simulink model "trajgen"  (Simulink 4.00)
settings: Solver=ode45  StartTime=0.0  StopTime=10.0  RelTol=1e-3
undefined symbols (not defined in the file or in its folder): nedaccel
settings Model: Creator=mcar  LastModifiedBy=mcar  BlockReductionOpt=off

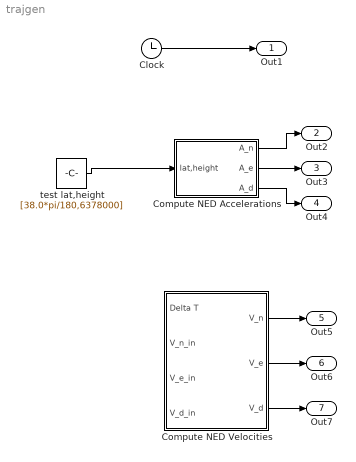
== system trajgen ==
  Clock : Clock
      settings: DisplayTime=off  Decimation=10
  Compute NED Accelerations : Subsystem
      settings: RTWFcnNameOpts=Auto  RTWFileNameOpts=Auto
  Compute NED Velocities : Subsystem
      settings: RTWFcnNameOpts=Auto  RTWFileNameOpts=Auto
  test lat,height : Constant  Value=[38.0*pi/180,6378000]  VectorParams1D=off
  Out1 : Outport  Port=1
  Out2 : Outport  Port=2
  Out3 : Outport  Port=3
  Out4 : Outport  Port=4
  Out5 : Outport  Port=5
  Out6 : Outport  Port=6
  Out7 : Outport  Port=7
  wires:
  Clock/1 -> Out1/1
  test lat,height/1 -> Compute NED Accelerations/1(lat,height)
  Compute NED Accelerations/3(A_d) -> Out4/1
  Compute NED Accelerations/2(A_e) -> Out3/1
  Compute NED Accelerations/1(A_n) -> Out2/1
  Compute NED Velocities/3(V_d) -> Out7/1
  Compute NED Velocities/2(V_e) -> Out6/1
  Compute NED Velocities/1(V_n) -> Out5/1

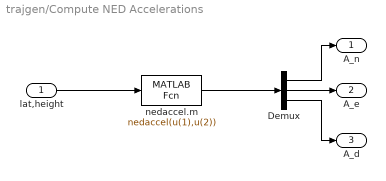
== system trajgen/Compute NED Accelerations ==
  lat,height : Inport  Port=1
  Demux : Demux  Outputs=3  BusSelectionMode=off
  nedaccel.m : MATLABFcn  MATLABFcn=nedaccel(u(1),u(2))  OutputDimensions=3  OutputSignalType=auto  Output1D=off
  A_n : Outport  Port=1
  A_e : Outport  Port=2
  A_d : Outport  Port=3
  wires:
  lat,height/1 -> nedaccel.m/1
  nedaccel.m/1 -> Demux/1
  Demux/1 -> A_n/1
  Demux/2 -> A_e/1
  Demux/3 -> A_d/1

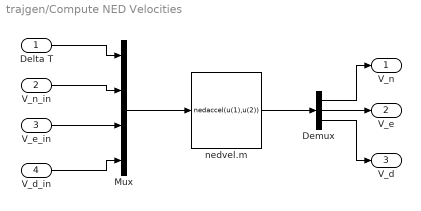
== system trajgen/Compute NED Velocities ==
  Delta T : Inport  Port=1
  V_n_in : Inport  Port=2
  V_e_in : Inport  Port=3
  V_d_in : Inport  Port=4
  Demux : Demux  Outputs=3  BusSelectionMode=off
  Mux : Mux  Inputs=4
  nedvel.m : MATLABFcn  MATLABFcn=nedaccel(u(1),u(2))  OutputDimensions=3  OutputSignalType=auto  Output1D=off
  V_n : Outport  Port=1
  V_e : Outport  Port=2
  V_d : Outport  Port=3
  wires:
  Demux/3 -> V_d/1
  Demux/2 -> V_e/1
  Demux/1 -> V_n/1
  nedvel.m/1 -> Demux/1
  Mux/1 -> nedvel.m/1
  V_d_in/1 -> Mux/4
  V_e_in/1 -> Mux/3
  V_n_in/1 -> Mux/2
  Delta T/1 -> Mux/1
